simulink model "baro_inertial"  (Simulink 5.0)
settings: Solver=ode45  StartTime=0.0  StopTime=3600  RelTol=1e-3
undefined symbols (not defined in the file or in its folder): plumbbobg
settings Model: Creator=mcarroll  LastModifiedBy=mcarroll  ExtModeAutoUpdateStatusClock=off

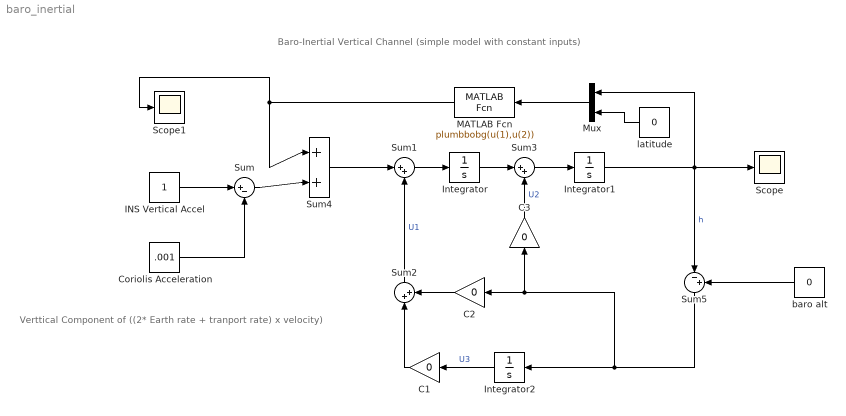
== system baro_inertial ==
  note: Baro-Inertial Vertical Channel
      | (simple model with constant inputs)
  note: Verttical Component of
      | ((2* Earth rate + tranport rate)
      | x velocity)
  C1 : Gain  Orientation=left  Gain=0  SaturateOnIntegerOverflow=on
  C2 : Gain  Orientation=left  Gain=0  SaturateOnIntegerOverflow=on
  C3 : Gain  Orientation=up  Gain=0  SaturateOnIntegerOverflow=on
  Coriolis Acceleration : Constant  Value=.001
  INS Vertical Accel : Constant
  Integrator : Integrator
  Integrator1 : Integrator
  Integrator2 : Integrator  Orientation=left
  MATLAB Fcn : MATLABFcn  Orientation=left  MATLABFcn=plumbbobg(u(1),u(2))
  Mux : Mux  Orientation=left  Inputs=2
  Scope : Scope
      settings: YMin=-8  YMax=8
  Scope1 : Scope
      settings: YMin=9.78859  YMax=9.78864
  Sum : Sum  Inputs=|+-  SaturateOnIntegerOverflow=on
  Sum1 : Sum  Inputs=|++  SaturateOnIntegerOverflow=on
  Sum2 : Sum  Orientation=up  Inputs=|++  SaturateOnIntegerOverflow=on
  Sum3 : Sum  Inputs=|++  SaturateOnIntegerOverflow=on
  Sum4 : Sum  Inputs=|++  SaturateOnIntegerOverflow=on
  Sum5 : Sum  Orientation=down  Inputs=|-+  SaturateOnIntegerOverflow=on
  baro alt : Constant  Orientation=left  Value=0
  latitude : Constant  Orientation=left  Value=0
  wires:
  baro alt/1 -> Sum5/2
  Integrator1/1 -> Sum5/1, Mux/1, Scope/1  "h"
  Sum5/1 -> Integrator2/1, C2/1, C3/1
  C3/1 -> Sum3/2  "U2"
  Integrator/1 -> Sum3/1
  Sum3/1 -> Integrator1/1
  Sum1/1 -> Integrator/1
  Sum4/1 -> Sum1/1
  Sum/1 -> Sum4/2
  MATLAB Fcn/1 -> Sum4/1, Scope1/1
  C2/1 -> Sum2/2
  Integrator2/1 -> C1/1  "U3"
  C1/1 -> Sum2/1
  Sum2/1 -> Sum1/2  "U1"
  Coriolis Acceleration/1 -> Sum/2
  INS Vertical Accel/1 -> Sum/1
  latitude/1 -> Mux/2
  Mux/1 -> MATLAB Fcn/1
